simulink library "fp_utilities_src"  (R2022b)
settings: Solver=VariableStepAuto  StartTime=0.0  StopTime=10.0  RelTol=1e-3
libraries: spsCurrentMeasurementLib x1, spsVoltageMeasurementLib x1
settings Model: Creator=Javnson  LastModifiedBy=javnson

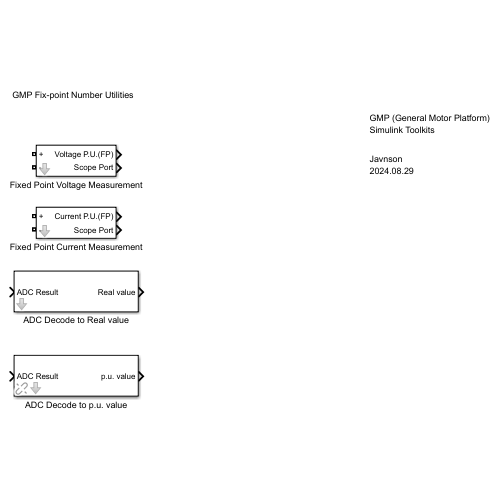
[thumbnail: Simulink's stored preview of the top-level diagram]
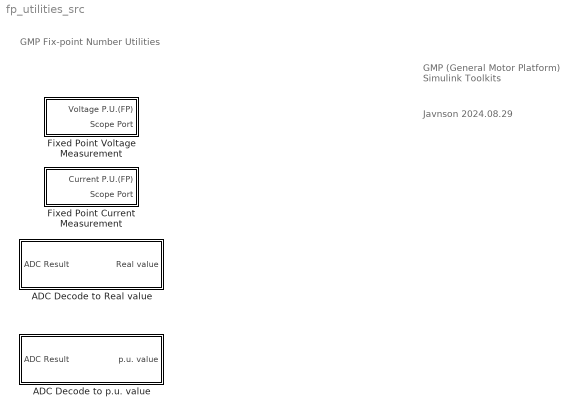
== system fp_utilities_src ==
  note: GMP Fix-point Number Utilities
  note: GMP (General Motor Platform)
      | Simulink Toolkits
  note: Javnson
      | 2024.08.29
  ADC Decode to Real value : Subsystem  mask{ADC_GAIN=1, ADC_BIT=16, ADC_REF=750, ADC_BIAS=385}
      settings: CopyFcn=set_param(gcbh,'LinkStatus','none');
      mask DialogControl DescGroupVar Prompt: ADC Decoder
      mask DialogControl DescTextVar Prompt: GMP CTL Simulink Utilities: virtual peripherals
      mask DialogControl Control2 Prompt: Transfer adc sample result to real value.
      mask DialogControl ParameterGroupVar Prompt: 参数
      mask DialogControl Control3 Prompt: ADC Voltage Gain (Scale Factor):
      mask DialogControl Control4 Prompt: ADC resolution:
      mask DialogControl Control5 Prompt: ADC reference Voltage (V), when ADC_GAIN=1, ADC_REF = ADC full scale
      mask DialogControl Control6 Prompt: ADC Bias Voltage(V)
  ADC Decode to p.u. value : Subsystem  AncestorBlock=fp_utilities/ADC Decode to Real value  mask{ADC_GAIN=1, ADC_BIT=16, ADC_REF=750, ADC_BIAS=385}
      settings: CopyFcn=set_param(gcbh,'LinkStatus','none');
      mask DialogControl DescGroupVar Prompt: ADC Decoder
      mask DialogControl DescTextVar Prompt: GMP CTL Simulink Utilities: virtual peripherals
      mask DialogControl Control2 Prompt: Transfer adc sample result to real value.
      mask DialogControl ParameterGroupVar Prompt: 参数
      mask DialogControl Control3 Prompt: ADC Voltage Gain (Scale Factor):
      mask DialogControl Control4 Prompt: ADC resolution:
      mask DialogControl Control5 Prompt: ADC reference Voltage (V), when ADC_GAIN=1, ADC_REF = ADC full scale
      mask DialogControl Control6 Prompt: ADC Bias Voltage(V)
  Fixed Point Current Measurement : Subsystem  mask{PerUnit_Base=60, Q_VALUE=24}
      mask prompts: PerUnit_Base "PerUnit_Base (A) :"; Q_VALUE "Q_num"
      settings: CopyFcn=set_param(gcbh,'LinkStatus','none');
      mask DialogControl DescGroupVar Prompt: Fixed Point Voltage Measurement
      mask DialogControl DescTextVar Prompt: Measure a voltage value and transfer the real value (double type) to perunit value(int32_t).
      mask DialogControl Control2 Prompt: Parameter per unit base value:
      mask DialogControl Control3 Prompt: Fixed-point Number Q value:
  Fixed Point Voltage Measurement : Subsystem  mask{PerUnit_Base=60, Q_VALUE=24}
      mask prompts: PerUnit_Base "PerUnit_Base (V) :"; Q_VALUE "Q_num"
      mask DialogControl DescGroupVar Prompt: Fixed Point Voltage Measurement
      mask DialogControl DescTextVar Prompt: Measure a voltage value and transfer the real value (double type) to perunit value(int32_t).
      mask DialogControl Control2 Prompt: Parameter per unit base value:
      mask DialogControl Control3 Prompt: Fixed-point Number Q value:

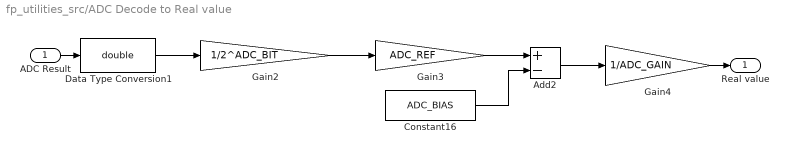
== system fp_utilities_src/ADC Decode to Real value ==
  ADC Result : Inport
  Add2 : Sum  Inputs=+-
  Constant16 : Constant  Value=ADC_BIAS
  Data Type Conversion1 : DataTypeConversion  OutDataTypeStr=double  SaturateOnIntegerOverflow=off  RndMeth=Floor
  Gain2 : Gain  Gain=1/2^ADC_BIT
  Gain3 : Gain  Gain=ADC_REF
  Gain4 : Gain  Gain=1/ADC_GAIN
  Real value : Outport
  wires:
  Data Type Conversion1/1 -> Gain2/1
  Gain3/1 -> Add2/1
  Add2/1 -> Gain4/1
  Gain4/1 -> Real value/1
  Constant16/1 -> Add2/2
  Gain2/1 -> Gain3/1
  ADC Result/1 -> Data Type Conversion1/1

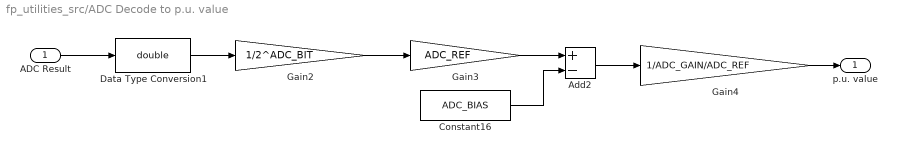
== system fp_utilities_src/ADC Decode to p.u. value ==
  ADC Result : Inport
  Add2 : Sum  Inputs=+-
  Constant16 : Constant  Value=ADC_BIAS
  Data Type Conversion1 : DataTypeConversion  OutDataTypeStr=double  SaturateOnIntegerOverflow=off  RndMeth=Floor
  Gain2 : Gain  Gain=1/2^ADC_BIT
  Gain3 : Gain  Gain=ADC_REF
  Gain4 : Gain  Gain=1/ADC_GAIN/ADC_REF
  p.u. value : Outport
  wires:
  Data Type Conversion1/1 -> Gain2/1
  Gain3/1 -> Add2/1
  Add2/1 -> Gain4/1
  Gain4/1 -> p.u. value/1
  Constant16/1 -> Add2/2
  Gain2/1 -> Gain3/1
  ADC Result/1 -> Data Type Conversion1/1

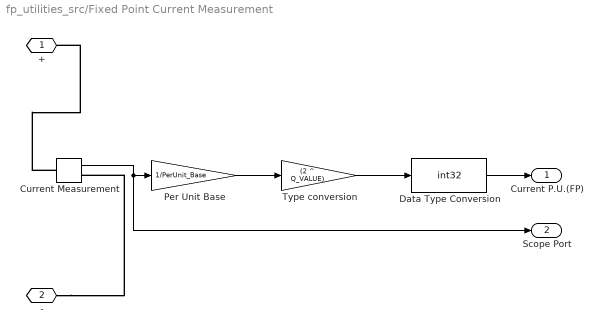
== system fp_utilities_src/Fixed Point Current Measurement ==
  Current Measurement : spsCurrentMeasurementLib/Current Measurement  PhasorSimulation=off  OutputType=Complex  PSBequivalent=0
  Data Type Conversion : DataTypeConversion  OutDataTypeStr=int32  ConvertRealWorld=Stored Integer (SI)  SaturateOnIntegerOverflow=off  RndMeth=Floor  LockScale=on
  Per Unit Base : Gain  Gain=1/PerUnit_Base
  Type conversion : Gain  Gain=(2 ^ Q_VALUE)
  + : PMIOPort  Side=Left
  - : PMIOPort  Port=2  Side=Left
  Current P.U.(FP) : Outport
  Scope Port : Outport  Port=2
  wires:
  Per Unit Base/1 -> Type conversion/1
  Type conversion/1 -> Data Type Conversion/1
  Data Type Conversion/1 -> Current P.U.(FP)/1
  Current Measurement/1 -> Scope Port/1, Per Unit Base/1
  connections:
  -/RConn1 -- Current Measurement/RConn1
  Current Measurement/LConn1 -- +/RConn1

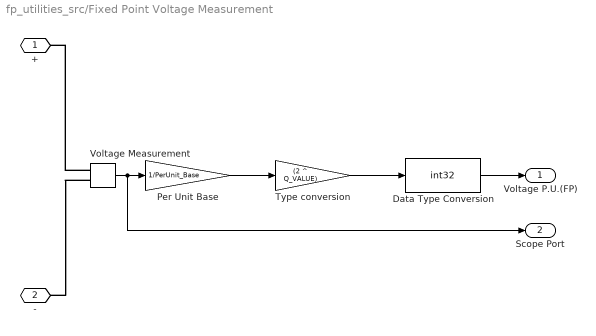
== system fp_utilities_src/Fixed Point Voltage Measurement ==
  Data Type Conversion : DataTypeConversion  OutDataTypeStr=int32  ConvertRealWorld=Stored Integer (SI)  SaturateOnIntegerOverflow=off  RndMeth=Floor  LockScale=on
  Per Unit Base : Gain  Gain=1/PerUnit_Base
  Type conversion : Gain  Gain=(2 ^ Q_VALUE)
  Voltage Measurement : spsVoltageMeasurementLib/Voltage Measurement  PhasorSimulation=off  OutputType=Complex  PSBequivalent=0
  + : PMIOPort  Side=Left
  - : PMIOPort  Port=2  Side=Left
  Voltage P.U.(FP) : Outport
  Scope Port : Outport  Port=2
  wires:
  Per Unit Base/1 -> Type conversion/1
  Type conversion/1 -> Data Type Conversion/1
  Data Type Conversion/1 -> Voltage P.U.(FP)/1
  Voltage Measurement/1 -> Scope Port/1, Per Unit Base/1
  connections:
  Voltage Measurement/LConn2 -- -/RConn1
  Voltage Measurement/LConn1 -- +/RConn1
